simulink model "TSPMe_cycle"  (R2023a)
settings: Solver=VariableStepAuto  StartTime=0.0  StopTime=10E5  FixedStep=1  RelTol=1e-3
libraries: fl_lib x8, nesl_utility x7, BatteryLibrary_lib x2
settings Model: Creator=widana_d  LastModifiedBy=widana_d
settings DataIOCC: SaveState=on
settings DebuggingCC: UnconnectedInputMsg=warning  UnconnectedOutputMsg=warning  UnconnectedLineMsg=warning
settings ModelReferenceCC: EnableRefExpFcnMdlSchedulingChecks=on
settings RTWCC: DLArmComputeVersion=19.05

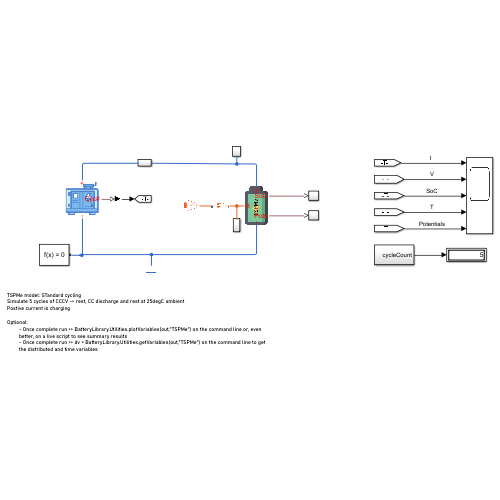
[thumbnail: Simulink's stored preview of the top-level diagram]
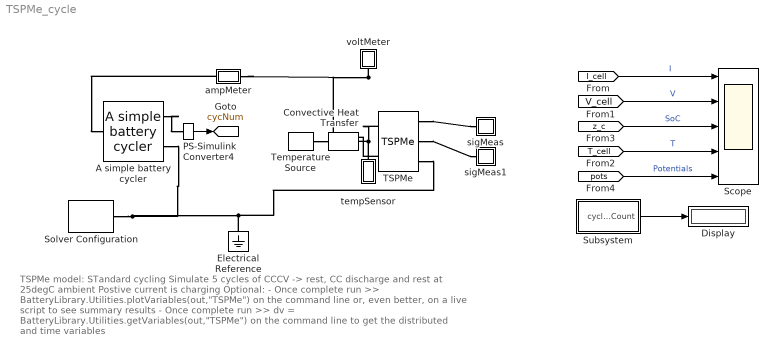
== system TSPMe_cycle ==
  note: TSPMe model: STandard cycling
      | Simulate 5 cycles of CCCV -> rest, CC discharge and rest at 25degC ambient
      | Postive current is charging
      |
      | Optional:
      | - Once complete run >> BatteryLibrary.Utilities.plotVariables(out,"TSPMe") on the command line or, even better, on a live script to see summary results
      | - Once complete run >> dv = BatteryLibrary.Utilities.getVariables(out,"TSPMe") on the command line to get the distributed and time variables
  A simple battery cycler : BatteryLibrary_lib/Utilities/A simple battery cycler  Vmax=4.2 V  Vmin=2.5 V  Ic=1.6 A  Ico=0.25 A  Id=-5 A  tRestC=1800 s  tRestD=3600 s
      settings: InternalSimscapePortConfiguration="{\"Bottom\":[{\"id\":\"n\",\"label\":\"-\",\"type\":\"foundation.electrical.electrical\"}],\"Left\":[],\"Right\":[{\"id\":\"numCyc\",\"label\":\"Cyc#\",\"type\":\"output\"}],\"Top\":[{\"id\":\"p\",\"label\":\"+\",\"type\":\"foundation.electrical.electrical\"}]}"
  Convective Heat Transfer : fl_lib/Thermal/Thermal Elements/Convective Heat Transfer  thermal_type=foundation.enum.constant_variable.constant  area=0.0046 m^2  heat_tr_coeff=35 W/(m^2 * K)  min_heat_tr_coeff=1e-3 W/(K*m^2)  T_specify=off  T_priority=None  T=0 K  T_nominal_specify=off  T_nominal_unit=K  T_nominal_value=1  Q_specify=off  Q_priority=None  Q=0 W  Q_nominal_specify=off  Q_nominal_unit=W  Q_nominal_value=1
  Display : Display
  Electrical Reference : fl_lib/Electrical/Electrical Elements/Electrical Reference
  PS-Simulink Converter4 : nesl_utility/PS-Simulink Converter  PhysicalDomain=network_engine_domain  SubClassName=ps_output  LeftPortType=input  RightPortType=output  PseudoPeriodic=off  Frequencies=[]  VectorFormat=1-D array  Unit=inherit  AffineConversion=off
  Scope : Scope  NumInputPorts=5
  Solver Configuration : nesl_utility/Solver Configuration  PhysicalDomain=network_engine_domain  SubClassName=solver  LeftPortType=input  RightPortType=generic  Tones=[]  Harmonics=[]  SimulateNoise=off  Profile=off  UseLocalSampling=off  EnableSwitchedLinearOptims=on  FrequencyDomain=off  UseCCode=off  RelTol=0.001  AbsTol=1e-06  MinStep=1e-09  ToWorkspace=off  RevertToSquareIcSolve=off  NumHomotopyIterations=100  PhasorMode=off  PhasorModeNumHarmonics=1  ConsistencySolver=NEWTON_FTOL  IndexReductionMethod=DerivativeReplacement  DoDC=off  ResidualTolerance=1e-09  ConsistencyTolSource=GLOBAL  ConsistencyAbsTol=0.001  ConsistencyRelTol=0.001  ConsistencyTolFactor=0.001  UseLocalSolver=off  LocalSolverChoice=NE_BACKWARD_EULER_ADVANCER  ResolveIndetEquations=on  FunctionEvalNumThread=1  LocalSolverSampleTime=0.001  DoFixedCost=off  MaxNonlinIter=3  MaxModeIter=2  ComputeImpulses=off  ImpulseIterations=2  LinearAlgebra=auto  LinearAlgebraNumThread=0  EquationFormulation=NE_TIME_EF  DelaysMemoryBudget=1024  AutomaticFiltering=on  FilteringTimeConstant=0.001  PartitionStorageMethod=AS_NEEDED  PartitionMemoryBudget=1024  PartitionMethod=ROBUST
  Subsystem : Subsystem
  TSPMe : BatteryLibrary_lib/Models/TSPMe  z0=0.5  T0=25 degC  Cn=4.9 hr*A  DnRef=3.3E-14 m^2/s  DpRef=4E-15 m^2/s  sigma_nRef=215 S/m  sigma_eRef=1.2 S/m  sigma_pRef=0.18 S/m  tr=0.2594  ce0=1000 mol/m^3  cn_max=33133 mol/m^3  cp_max=63104 mol/m^3  sn_max=0.9014  sn_min=0.0279  sp_max=0.9072  sp_min=0.2567  knRef=6.48E-7 m^2.50000*A/mol^1.50000  kpRef=3.42E-6 m^2.50000*A/mol^1.50000  Cp=110 J/K  Tref=298 K  Ea_kn=1 kJ/mol  Ea_kp=1 kJ/mol  Ea_Dn=75 kJ/mol  Ea_Dp=10 kJ/mol  Ea_De=1.2 kJ/mol  Ea_sigman=80 kJ/mol  Ea_sigmae=80 kJ/mol  Ea_sigmap=80 kJ/mol  Ln=85.2 um  Ls=12 um  Lp=75.6 um  Area_p=1027 cm^2  eps_n=0.25  eps_s=0.47  eps_p=0.335  Rn=5.86 um  Rp=5.22 um  an=3.84E5 1/m  ap=3.82E5 1/m
      settings: InternalSimscapePortConfiguration="{\"Bottom\":[{\"id\":\"n\",\"label\":\"-\",\"type\":\"foundation.electrical.electrical\"}],\"Left\":[{\"id\":\"Hi\",\"label\":\"H\",\"type\":\"foundation.thermal.thermal\"}],\"Right\":[{\"id\":\"z\",\"label\":\"SoC\",\"type\":\"output\"},{\"id\":\"pots\",\"label\":\"Pots\",\"type\":\"output\"}],\"Top\":[{\"id\":\"p\",\"label\":\"+\",\"type\":\"foundation.electrical.electrical\"}]}"
  Temperature Source : fl_lib/Thermal/Thermal Sources/Temperature Source  temperature=25 degC
  ampMeter : Subsystem
  sigMeas : Subsystem
  sigMeas1 : Subsystem
  tempSensor : Subsystem
  voltMeter : Subsystem
  tag scope: cycNum=global
  wires:
  [V_cell] -> Scope/2  "V"
  [z_c] -> Scope/3  "SoC"
  [T_cell] -> Scope/4  "T"
  PS-Simulink Converter4/1 -> [cycNum]
  Subsystem/1(cycleCount) -> Display/1
  [I_cell] -> Scope/1  "I"
  [pots] -> Scope/5  "Potentials"
  connections:
  ampMeter/RConn1 -- TSPMe/LConn2 -- voltMeter/LConn1
  Solver Configuration/RConn1 -- A simple battery cycler/RConn2 -- TSPMe/RConn3 -- Electrical Reference/LConn1
  tempSensor/LConn1 -- TSPMe/LConn1 -- Convective Heat Transfer/LConn1
  Temperature Source/LConn1 -- Convective Heat Transfer/RConn1
  ampMeter/LConn1 -- A simple battery cycler/LConn1
  A simple battery cycler/RConn1 -- PS-Simulink Converter4/LConn1
  TSPMe/RConn1 -- sigMeas/LConn1
  TSPMe/RConn2 -- sigMeas1/LConn1

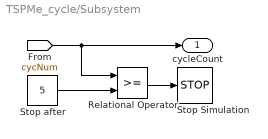
== system TSPMe_cycle/Subsystem ==
  Relational Operator : RelationalOperator  OutDataTypeStr=boolean  RndMeth=Simplest  InputSameDT=off
  Stop Simulation : Stop
  Stop after : Constant  Value=5
  cycleCount : Outport
  wires:
  Stop after/1 -> Relational Operator/2
  [cycNum] -> Relational Operator/1, cycleCount/1
  Relational Operator/1 -> Stop Simulation/1

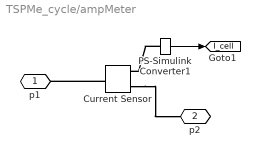
== system TSPMe_cycle/ampMeter ==
  Current Sensor : fl_lib/Electrical/Electrical Sensors/Current Sensor
  PS-Simulink Converter1 : nesl_utility/PS-Simulink Converter  PhysicalDomain=network_engine_domain  SubClassName=ps_output  LeftPortType=input  RightPortType=output  PseudoPeriodic=off  Frequencies=[]  VectorFormat=1-D array  Unit=inherit  AffineConversion=off
  p1 : PMIOPort  Side=Left
  p2 : PMIOPort  Port=2  Side=Right
  tag scope: I_cell=global
  wires:
  PS-Simulink Converter1/1 -> [I_cell]
  connections:
  Current Sensor/RConn2 -- p2/RConn1
  Current Sensor/LConn1 -- p1/RConn1
  PS-Simulink Converter1/LConn1 -- Current Sensor/RConn1

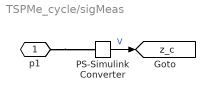
== system TSPMe_cycle/sigMeas ==
  PS-Simulink Converter : nesl_utility/PS-Simulink Converter  PhysicalDomain=network_engine_domain  SubClassName=ps_output  LeftPortType=input  RightPortType=output  PseudoPeriodic=off  Frequencies=[]  VectorFormat=1-D array  Unit=inherit  AffineConversion=off
  p1 : PMIOPort  Side=Left
  tag scope: z_c=global
  wires:
  PS-Simulink Converter/1 -> [z_c]  "V"
  connections:
  p1/RConn1 -- PS-Simulink Converter/LConn1

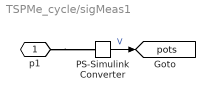
== system TSPMe_cycle/sigMeas1 ==
  PS-Simulink Converter : nesl_utility/PS-Simulink Converter  PhysicalDomain=network_engine_domain  SubClassName=ps_output  LeftPortType=input  RightPortType=output  PseudoPeriodic=off  Frequencies=[]  VectorFormat=1-D array  Unit=inherit  AffineConversion=off
  p1 : PMIOPort  Side=Left
  tag scope: pots=global
  wires:
  PS-Simulink Converter/1 -> [pots]  "V"
  connections:
  p1/RConn1 -- PS-Simulink Converter/LConn1

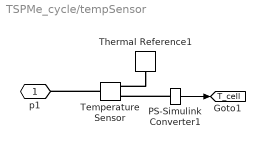
== system TSPMe_cycle/tempSensor ==
  PS-Simulink Converter1 : nesl_utility/PS-Simulink Converter  PhysicalDomain=network_engine_domain  SubClassName=ps_output  LeftPortType=input  RightPortType=output  PseudoPeriodic=off  Frequencies=[]  VectorFormat=1-D array  Unit=inherit  AffineConversion=off
  Temperature Sensor : fl_lib/Thermal/Thermal Sensors/Temperature Sensor  temperature_measure=foundation.enum.MeasurementReference.difference
  Thermal Reference1 : fl_lib/Thermal/Thermal Elements/Thermal Reference
  p1 : PMIOPort  Side=Left
  tag scope: T_cell=global
  wires:
  PS-Simulink Converter1/1 -> [T_cell]
  connections:
  Temperature Sensor/LConn1 -- p1/RConn1
  PS-Simulink Converter1/LConn1 -- Temperature Sensor/RConn2
  Thermal Reference1/LConn1 -- Temperature Sensor/RConn1

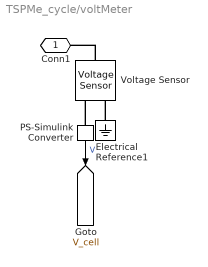
== system TSPMe_cycle/voltMeter ==
  Electrical Reference1 : fl_lib/Electrical/Electrical Elements/Electrical Reference
  PS-Simulink Converter : nesl_utility/PS-Simulink Converter  PhysicalDomain=network_engine_domain  SubClassName=ps_output  LeftPortType=input  RightPortType=output  PseudoPeriodic=off  Frequencies=[]  VectorFormat=1-D array  Unit=inherit  AffineConversion=off
  Voltage Sensor : fl_lib/Electrical/Electrical Sensors/Voltage Sensor
  Conn1 : PMIOPort  Side=Left
  tag scope: V_cell=global
  wires:
  PS-Simulink Converter/1 -> [V_cell]  "V"
  connections:
  Voltage Sensor/LConn1 -- Conn1/RConn1
  PS-Simulink Converter/LConn1 -- Voltage Sensor/RConn1
  Electrical Reference1/LConn1 -- Voltage Sensor/RConn2
